simulink model "S_RCL"  (R2024b)
settings: Solver=ode23  StartTime=0.0  StopTime=0.01  RelTol=1e-3
model workspace (MAT data in the model file):
  C = 1e-07
  L = 0.004
  R = 120
settings Model: Creator=DELL  LastModifiedBy=DELL

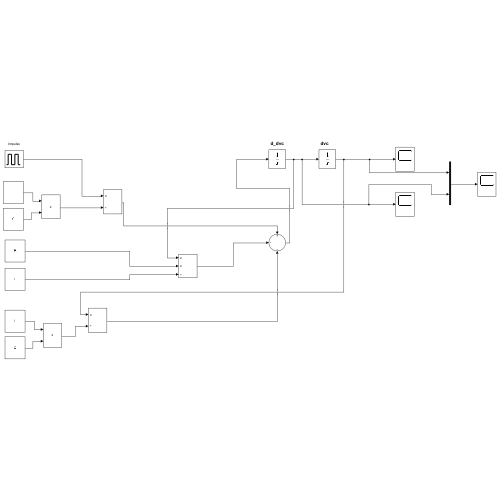
[thumbnail: Simulink's stored preview of the top-level diagram]
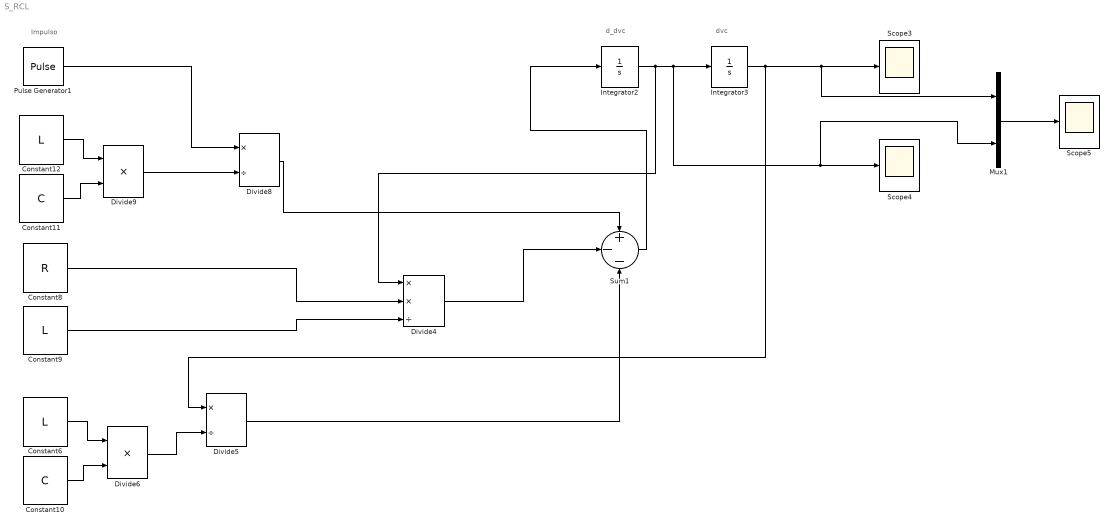
== system S_RCL ==
  note: Impulso
  note: d_dvc
  note: dvc
  Constant10 : Constant  Value=C
  Constant11 : Constant  Value=C
  Constant12 : Constant  Value=L
  Constant6 : Constant  Value=L
  Constant8 : Constant  Value=R
  Constant9 : Constant  Value=L
  Divide4 : Product  Inputs=**/
  Divide5 : Product  Inputs=*/
  Divide6 : Product  Inputs=**
  Divide8 : Product  Inputs=*/
  Divide9 : Product  Inputs=**
  Integrator2 : Integrator
  Integrator3 : Integrator
  Mux1 : Mux  Inputs=2
  Pulse Generator1 : DiscretePulseGenerator  PulseType=Time based  Amplitude=5  Period=2e-3  PulseWidth=50%
  Scope3 : Scope
  Scope4 : Scope
  Scope5 : Scope
  Sum1 : Sum  Inputs=+--
  wires:
  Constant10/1 -> Divide6/2
  Integrator2/1 -> Mux1/2, Scope4/1, Integrator3/1, Divide4/1
  Sum1/1 -> Integrator2/1
  Constant9/1 -> Divide4/3
  Divide6/1 -> Divide5/2
  Divide5/1 -> Sum1/3
  Constant8/1 -> Divide4/2
  Divide4/1 -> Sum1/2
  Integrator3/1 -> Mux1/1, Scope3/1, Divide5/1
  Mux1/1 -> Scope5/1
  Constant6/1 -> Divide6/1
  Divide8/1 -> Sum1/1
  Divide9/1 -> Divide8/2
  Constant11/1 -> Divide9/2
  Constant12/1 -> Divide9/1
  Pulse Generator1/1 -> Divide8/1
